simulink model "s_c107m32k_vlbi"  (R2018a)
settings: Solver=VariableStepDiscrete  StartTime=0.0  StopTime=(2^15)*10  RelTol=1e-3
undefined symbols (not defined in the file): fft_stages, n_bits_xengs
libraries: xbsIndex_r4 x23049, casper_library_misc x45, xps_library x4, casper_library_scopes x3, simulink x2
(part 44 of 201)

== system s_c107m32k_vlbi/bs_delay1/bus_expand1 ==
  bus_in : Inport
  reinterpret1 : xbsIndex_r4/Reinterpret  force_arith_type=on  arith_type="Signed  (2's comp)"  force_bin_pt=on  bin_pt=31  block_type=reinterpret
  reinterpret2 : xbsIndex_r4/Reinterpret  force_arith_type=on  arith_type="Signed  (2's comp)"  force_bin_pt=on  bin_pt=31  block_type=reinterpret
  reinterpret3 : xbsIndex_r4/Reinterpret  force_arith_type=on  arith_type="Signed  (2's comp)"  force_bin_pt=on  bin_pt=31  block_type=reinterpret
  reinterpret4 : xbsIndex_r4/Reinterpret  force_arith_type=on  arith_type=Unsigned  force_bin_pt=on  bin_pt=32  block_type=reinterpret
  slice1 : xbsIndex_r4/Slice  nbits=32  boolean_output=off  mode=Upper Bit Location + Width  bit1=-128  base1=MSB of Input  bit0=0  base0=LSB of Input  dbl_ovrd=off  block_type=slice
  slice2 : xbsIndex_r4/Slice  nbits=32  boolean_output=off  mode=Upper Bit Location + Width  bit1=-96  base1=MSB of Input  bit0=0  base0=LSB of Input  dbl_ovrd=off  block_type=slice
  slice3 : xbsIndex_r4/Slice  nbits=32  boolean_output=off  mode=Upper Bit Location + Width  bit1=-64  base1=MSB of Input  bit0=0  base0=LSB of Input  dbl_ovrd=off  block_type=slice
  slice4 : xbsIndex_r4/Slice  nbits=64  boolean_output=off  mode=Upper Bit Location + Width  bit1=0  base1=MSB of Input  bit0=0  base0=LSB of Input  dbl_ovrd=off  block_type=slice
  msb_out4 : Outport
  out3 : Outport  Port=2
  out2 : Outport  Port=3
  lsb_out1 : Outport  Port=4
  wires:
  reinterpret1/1 -> lsb_out1/1
  slice1/1 -> reinterpret1/1
  reinterpret2/1 -> out2/1
  slice2/1 -> reinterpret2/1
  reinterpret3/1 -> out3/1
  slice3/1 -> reinterpret3/1
  reinterpret4/1 -> msb_out4/1
  slice4/1 -> reinterpret4/1
  bus_in/1 -> slice1/1, slice2/1, slice3/1, slice4/1

== system s_c107m32k_vlbi/bs_delay1/delay_gen ==
  note: coarse delay rotates phase around 0th
      | channel. We want to reference with respect to
      | centre of band. So subtract half the coarse
      | delay amount.
  note: Extract fractional part
  note: Extract whole part
  note: Need negative slope
      | for positive deay
  note: Make space here (cast) for the upcoming
      | scaling, ensuring that we keep the
      | required precision.
      | Shift phase and delay rates down
      | to fit into specified range.
      | An update is only done at the end of
      | every FFT spectrum so modify shift to
      | not be as large
  sync_in : Inport
  init : Inport  Port=2
  din : Inport  Port=3
  idx_in : Inport  Port=4
  den : Inport  Port=5
  load : Inport  Port=6
  phase : Inport  Port=7
  d/dt_phase : Inport  Port=8
  delay : Inport  Port=9
  d/dt_delay : Inport  Port=10
  invert_slope : Inport  Port=11
  AddSub : xbsIndex_r4/AddSub  mode=Addition  use_carryin=off  use_carryout=off  en=off  latency=1  precision=Full  arith_type=Unsigned  n_bits=16  bin_pt=14  quantization=Truncate  overflow=Wrap  use_behavioral_HDL=on  hw_selection=Fabric  pipelined=off  dbl_ovrd=off  block_type=addsub
  Concat : xbsIndex_r4/Concat  num_inputs=4  dbl_ovrd=off  block_type=concat
  Constant : xbsIndex_r4/Constant  const=1  gui_display_data_type=Fixed-point  arith_type=Unsigned  n_bits=1  bin_pt=0  preci_type=Single  exp_width=8  frac_width=24  explicit_period=on  period=1  equ=P=C  opselect=C  inp2=PCIN>>17  opr=+  inp1=P  carry=CIN  dbl_ovrd=off  block_type=constant
  Convert : xbsIndex_r4/Convert  gui_display_data_type=Fixed-point  arith_type="Signed  (2's comp)"  n_bits=comp_phase_rate_bits  bin_pt=comp_phase_rate_bin_pt  float_type=Single  exp_bits=8  fraction_bits=24  quantization="Round  (unbiased: +/- Inf)"  overflow=Saturate  en=off  latency=0  pipeline=off  dbl_ovrd=off  block_type=convert
  Convert1 : xbsIndex_r4/Convert  gui_display_data_type=Fixed-point  arith_type="Signed  (2's comp)"  n_bits=comp_delay_rate_bits  bin_pt=comp_delay_rate_bin_pt  float_type=Single  exp_bits=8  fraction_bits=24  quantization="Round  (unbiased: +/- Inf)"  overflow=Saturate  en=off  latency=0  pipeline=off  dbl_ovrd=off  block_type=convert
  Convert4 : xbsIndex_r4/Convert  gui_display_data_type=Fixed-point  arith_type="Signed  (2's comp)"  n_bits=max(phase_bits, comp_phase_rate_bits)  bin_pt=max(phase_bits-1, comp_phase_rate_bin_pt)  float_type=Single  exp_bits=8  fraction_bits=24  quantization=Truncate  overflow=Wrap  en=off  latency=1  pipeline=on  dbl_ovrd=off  block_type=convert
      settings: block_version=10.1.3
  Convert5 : xbsIndex_r4/Convert  gui_display_data_type=Fixed-point  arith_type=Unsigned  n_bits=cd_bits  bin_pt=0  float_type=Single  exp_bits=8  fraction_bits=24  quantization=Truncate  overflow=Wrap  en=off  latency=1  pipeline=on  dbl_ovrd=off  block_type=convert
      settings: block_version=10.1.3
  Convert6 : xbsIndex_r4/Convert  gui_display_data_type=Fixed-point  arith_type=Unsigned  n_bits=max(delay_bin_pt, comp_delay_rate_bin_pt)  bin_pt=max(delay_bin_pt, comp_delay_rate_bin_pt)  float_type=Single  exp_bits=8  fraction_bits=24  quantization=Truncate  overflow=Wrap  en=off  latency=1  pipeline=on  dbl_ovrd=off  block_type=convert
      settings: block_version=10.1.3
  Delay{1..14,16} (15 alike) : xbsIndex_r4/Delay  rst=off  infoeditControl=Selection of Reset will increase slice count due to use of real FFs and instead of SRLs  en=off  latency=1  reg_retiming=on  dbl_ovrd=off  block_type=delay
      settings: block_version=11.4
  Mux : xbsIndex_r4/Mux  inputs=2  en=off  latency=1  precision=Full  arith_type=Unsigned  n_bits=16  bin_pt=14  quantization=Truncate  overflow=Wrap  dbl_ovrd=off  block_type=mux
      settings: block_version=11.4
  Negate : xbsIndex_r4/Negate  precision=Full  arith_type="Signed  (2's comp)"  n_bits=lookup_bits + fft_len  bin_pt=lookup_bits + fft_len - 1  quantization=Truncate  overflow=Saturate  en=off  latency=1  dbl_ovrd=off  block_type=negate
      settings: block_version=11.4
  Reinterpret{,1..3} (4 alike) : xbsIndex_r4/Reinterpret  force_arith_type=on  arith_type=Unsigned  force_bin_pt=on  bin_pt=0  block_type=reinterpret
  Slice5 : xbsIndex_r4/Slice  nbits=2  boolean_output=off  mode=Lower Bit Location + Width  bit1=0  base1=MSB of Input  bit0=0  base0=LSB of Input  dbl_ovrd=off  block_type=slice
  Terminator : Terminator
  Terminator1 : Terminator
  bus_expand : Subsystem  AncestorBlock=casper_library_flow_control/bus_expand  mask(bus_expand){mode=divisions of arbitrary size, outputNum=1, outputWidth=[1 1 data_bits n_bits_index], outputBinaryPt=[0 0 0 0], outputArithmeticType=[2 2 0 0], show_format=off, outputToWorkspace=off, variablePrefix=out, outputToModelAsWell=on}
      mask prompts: outputNum "Number of outputs:"; outputWidth "Output width [msb ... lsb]:"; outputBinaryPt "Output binary point position [msb ... lsb]:"; outputArithmeticType "Output arithmetic type (ufix=0, fix=1, bool=2) [msb ... lsb]:"; show_format "Print format string?"; outputToWorkspace "Output to workspace?"; variablePrefix "Variable name prefix:"; outputToModelAsWell "Output to model as well?"
      mask help:
      | Expands a 'bus' made using a bus_create or Xilinx
      | concat block.
      | The input will be divided into the specified number
      | of outputs with the specified arithmetic types.
      | Divisions are made from most significant bit.
      mask init: same as s_c107m32k_vlbi/bus_expand1
      settings: AttributesFormatString=4 outputs
      mask TypeOptions mode: divisions of equal size | divisions of arbitrary size
      mask Callback mode: bus_expand_callback();
      mask Callback outputWidth: bus_expand_callback();
      mask Callback outputToWorkspace: bus_expand_callback();
  delay_calc : Subsystem  mask{bit_width=max(delay_bits, comp_delay_rate_bits), bin_pt=max(delay_bin_pt, comp_delay_rate_bin_pt)}
      mask prompts: bit_width "Coefficient bit width"; bin_pt "Coefficient binary point"
  half_cd : xbsIndex_r4/Shift  shift_dir=Right  shift_bits=1  en=off  latency=0  precision=User Defined  arith_type=Unsigned  n_bits=2  bin_pt=1  quantization=Truncate  overflow=Saturate  dbl_ovrd=off  block_type=shift
  normalise+fft0 : xbsIndex_r4/Shift  shift_dir=Right  shift_bits=phase_rate_scale_factor  en=off  latency=0  precision=Full  arith_type="Signed  (2's comp)"  n_bits=comp_phase_rate_bits  bin_pt=comp_phase_rate_bin_pt  quantization="Round  (unbiased: +/- Inf)"  overflow=Saturate  dbl_ovrd=off  block_type=shift
  normalise+fft1 : xbsIndex_r4/Shift  shift_dir=Right  shift_bits=delay_rate_scale_factor  en=off  latency=0  precision=Full  arith_type="Signed  (2's comp)"  n_bits=comp_delay_rate_bits  bin_pt=comp_delay_rate_bin_pt  quantization="Round  (unbiased: +/- Inf)"  overflow=Saturate  dbl_ovrd=off  block_type=shift
  phase_calc : Subsystem  mask{bit_width=max(phase_bits, comp_phase_rate_bits), bin_pt=max(phase_bits-1, comp_phase_rate_bin_pt)}
      mask prompts: bit_width "Coefficient bit width"; bin_pt "Coefficient binary point"
  sync_out : Outport
  dout : Outport  Port=2
  idx_out : Outport  Port=3
  dvalid : Outport  Port=4
  cd_o : Outport  Port=5
  slope_out : Outport  Port=6
  phase_out : Outport  Port=7
  load_out : Outport  Port=8
  wires:
  Convert1/1 -> normalise+fft1/1
  Convert/1 -> normalise+fft0/1
  Delay14/1 -> cd_o/1
  Delay10/1 -> phase_out/1
  Delay7/1 -> load_out/1
  Delay6/1 -> bus_expand/1(bus_in)
  bus_expand/4(lsb_out1) -> idx_out/1
  bus_expand/3(out2) -> dout/1
  bus_expand/2(out3) -> dvalid/1
  idx_in/1 -> Reinterpret3/1
  din/1 -> Reinterpret2/1
  den/1 -> Reinterpret1/1
  bus_expand/1(msb_out4) -> sync_out/1
  Reinterpret3/1 -> Concat/4
  Reinterpret2/1 -> Concat/3
  Reinterpret1/1 -> Concat/2
  Reinterpret/1 -> Concat/1
  Delay13/1 -> Mux/3
  delay_calc/1(dout) -> Terminator1/1
  Constant/1 -> delay_calc/1(din)
  delay/1 -> delay_calc/2(val)
  phase/1 -> phase_calc/2(val)
  Delay12/1 -> Convert6/1
  Delay11/1 -> Delay8/1
  Delay3/1 -> AddSub/1
  Delay1/1 -> Delay4/1
  Delay9/1 -> Delay6/1
  phase_calc/1(dout) -> Delay11/1
  AddSub/1 -> Convert4/1
  phase_calc/2(coeff) -> Delay3/1
  half_cd/1 -> AddSub/2
  Slice5/1 -> half_cd/1
  Convert5/1 -> Delay5/1, Slice5/1
  Concat/1 -> phase_calc/1(din)
  sync_in/1 -> Reinterpret/1
  init/1 -> [tick]
  Delay8/1 -> Delay9/1
  Negate/1 -> Mux/2
  invert_slope/1 -> Mux/1
  Delay5/1 -> Delay16/1
  Delay4/1 -> Delay2/1
  load/1 -> [en]
  normalise+fft0/1 -> phase_calc/3(val_inc)
  [en] -> phase_calc/4(en)
  [en] -> delay_calc/4(en)
  [tick] -> phase_calc/5(update)
  [tick] -> delay_calc/5(update)
  delay_calc/2(coeff) -> Convert5/1, Delay12/1
  phase_calc/3(en_o) -> Delay1/1
  delay_calc/3(en_o) -> Terminator/1
  Convert6/1 -> Negate/1, Delay13/1
  Mux/1 -> slope_out/1
  Convert4/1 -> Delay10/1
  Delay2/1 -> Delay7/1
  Delay16/1 -> Delay14/1
  d/dt_phase/1 -> Convert/1
  normalise+fft1/1 -> delay_calc/3(val_inc)
  d/dt_delay/1 -> Convert1/1

== system s_c107m32k_vlbi/bs_delay1/edge_detect ==
  in : Inport
  Delay : xbsIndex_r4/Delay  rst=off  infoeditControl=Selection of Reset will increase slice count due to use of real FFs and instead of SRLs  en=off  latency=1  reg_retiming=off  dbl_ovrd=off  block_type=delay
      settings: xl_area=[0, 0, 0, 0, 0, 0, 0]
  Inverter : xbsIndex_r4/Inverter  en=off  latency=0  dbl_ovrd=off  block_type=inv
      settings: xl_area=[0, 0, 0, 0, 0, 0, 0]
  edge_op : xbsIndex_r4/Logical  logical_function=NOR  inputs=2  en=off  latency=0  precision=Full  arith_type=Unsigned  n_bits=8  bin_pt=2  align_bp=on  dbl_ovrd=off  block_type=logical
      settings: xl_area=[0, 0, 0, 0, 0, 0, 0]
  out : Outport
  wires:
  Delay/1 -> edge_op/2
  in/1 -> Delay/1, Inverter/1
  edge_op/1 -> out/1
  Inverter/1 -> edge_op/1

== system s_c107m32k_vlbi/bs_delay1/generate_pkt_sync1 ==
  sync : Inport
  valid : Inport  Port=2
  data : Inport  Port=3
  Constant : xbsIndex_r4/Constant  const=(2^pktlen_bits)-1  gui_display_data_type=Fixed-point  arith_type=Unsigned  n_bits=pktlen_bits  bin_pt=0  preci_type=Single  exp_width=8  frac_width=24  explicit_period=on  period=1  equ=P=C  opselect=C  inp2=PCIN>>17  opr=+  inp1=P  carry=CIN  dbl_ovrd=off  block_type=constant
  Counter1 : xbsIndex_r4/Counter  cnt_type=Free Running  cnt_to=Inf  operation=Up  start_count=0  cnt_by_val=1  arith_type=Unsigned  n_bits=pktlen_bits  bin_pt=0  load_pin=off  rst=on  en=on  explicit_period=on  period=1  use_behavioral_HDL=on  implementation=Fabric  dbl_ovrd=off  block_type=counter
  Delay{,1..5} (6 alike) : xbsIndex_r4/Delay  rst=off  infoeditControl=Selection of Reset will increase slice count due to use of real FFs and instead of SRLs  en=off  latency=1  reg_retiming=on  dbl_ovrd=off  block_type=delay
  Logical : xbsIndex_r4/Logical  logical_function=OR  inputs=2  en=off  latency=1  precision=Full  arith_type=Unsigned  n_bits=16  bin_pt=0  align_bp=on  dbl_ovrd=off  block_type=logical
  Logical1 : xbsIndex_r4/Logical  logical_function=AND  inputs=2  en=off  latency=0  precision=Full  arith_type=Unsigned  n_bits=16  bin_pt=0  align_bp=on  dbl_ovrd=off  block_type=logical
  Relational : xbsIndex_r4/Relational  mode=a=b  op_type=Bool  en=off  latency=1  dbl_ovrd=off  block_type=relational
  pipeline1 : Subsystem  Tag=cmac_delinked  mask(pipeline){csp_latency=2}
      mask prompts: csp_latency "Latency"
      mask help:
      | An explicitly laid-out delay line to avoid mapping to SRL16s
      | for use in pipelining to help achieve timing closure.
      mask init:
      | pipeline_init(gcb,'latency',csp_latency);
      settings: AttributesFormatString=Latency = %<latency>
      mask Display:
      | port_label('input', 1, 'd');
      | port_label('output', 1, 'q');
      | disp(['Z^-', num2str(csp_latency)]);
  pipeline2 : Subsystem  Tag=cmac_delinked  mask(pipeline){csp_latency=2}
      mask prompts: csp_latency "Latency"
      mask help:
      | An explicitly laid-out delay line to avoid mapping to SRL16s
      | for use in pipelining to help achieve timing closure.
      mask init:
      | pipeline_init(gcb,'latency',csp_latency);
      settings: AttributesFormatString=Latency = %<latency>
      mask Display:
      | port_label('input', 1, 'd');
      | port_label('output', 1, 'q');
      | disp(['Z^-', num2str(csp_latency)]);
  pipeline24 : Subsystem  Tag=cmac_delinked  mask(pipeline){csp_latency=2}
      mask prompts: csp_latency "Latency"
      mask help:
      | An explicitly laid-out delay line to avoid mapping to SRL16s
      | for use in pipelining to help achieve timing closure.
      mask init:
      | pipeline_init(gcb,'latency',csp_latency);
      settings: AttributesFormatString=Latency = %<latency>
      mask Display:
      | port_label('input', 1, 'd');
      | port_label('output', 1, 'q');
      | disp(['Z^-', num2str(csp_latency)]);
  out_sync : Outport
  out_valid : Outport  Port=2
  out_data : Outport  Port=3
  packet_sync : Outport  Port=4
  wires:
  Delay5/1 -> Logical1/1, Delay/1
  Delay4/1 -> Delay1/1, Logical/1
  Delay3/1 -> Delay2/1
  Logical/1 -> packet_sync/1
  Delay/1 -> out_valid/1
  Delay1/1 -> out_sync/1
  Delay2/1 -> out_data/1
  pipeline2/1(q) -> Counter1/1, Delay4/1
  pipeline1/1(q) -> Counter1/2, Delay5/1
  pipeline24/1(q) -> Delay3/1
  data/1 -> pipeline24/1(d)
  valid/1 -> pipeline1/1(d)
  sync/1 -> pipeline2/1(d)
  Logical1/1 -> Logical/2  "ns"
  Relational/1 -> Logical1/2
  Constant/1 -> Relational/2
  Counter1/1 -> Relational/1  "pkt_counter"

== system s_c107m32k_vlbi/bs_delay1/mangled_dwp ==
  note: JRM: customised block
      | Replaced BRAM delays
      | with distributed memory.
      | THIS BLOCK IS NO LONGER PROPERLY PARAMETERISED!
  sync : Inport
  delay : Inport  Port=2
  ld_delay : Inport  Port=3
  data_in0 : Inport  Port=4
  data_in1 : Inport  Port=5
  data_in2 : Inport  Port=6
  data_in3 : Inport  Port=7
  data_in4 : Inport  Port=8
  data_in5 : Inport  Port=9
  data_in6 : Inport  Port=10
  data_in7 : Inport  Port=11
  en : Inport  Port=12
  AddSub{1..7} (7 alike) : xbsIndex_r4/AddSub  mode=Addition  use_carryin=off  use_carryout=off  en=off  latency=0  precision=Full  arith_type=Unsigned  n_bits=1  bin_pt=0  quantization=Truncate  overflow=Wrap  use_behavioral_HDL=off  hw_selection=Fabric  pipelined=off  dbl_ovrd=off  block_type=addsub
  Constant1 : xbsIndex_r4/Constant  const=6  gui_display_data_type=Fixed-point  arith_type=Unsigned  n_bits=3  bin_pt=0  preci_type=Single  exp_width=8  frac_width=24  explicit_period=on  period=1  equ=P=C  opselect=C  inp2=PCIN>>17  opr=+  inp1=P  carry=CIN  dbl_ovrd=off  block_type=constant
  Constant2 : xbsIndex_r4/Constant  const=5  gui_display_data_type=Fixed-point  arith_type=Unsigned  n_bits=3  bin_pt=0  preci_type=Single  exp_width=8  frac_width=24  explicit_period=on  period=1  equ=P=C  opselect=C  inp2=PCIN>>17  opr=+  inp1=P  carry=CIN  dbl_ovrd=off  block_type=constant
  Constant3 : xbsIndex_r4/Constant  const=4  gui_display_data_type=Fixed-point  arith_type=Unsigned  n_bits=3  bin_pt=0  preci_type=Single  exp_width=8  frac_width=24  explicit_period=on  period=1  equ=P=C  opselect=C  inp2=PCIN>>17  opr=+  inp1=P  carry=CIN  dbl_ovrd=off  block_type=constant
  Constant4 : xbsIndex_r4/Constant  const=3  gui_display_data_type=Fixed-point  arith_type=Unsigned  n_bits=3  bin_pt=0  preci_type=Single  exp_width=8  frac_width=24  explicit_period=on  period=1  equ=P=C  opselect=C  inp2=PCIN>>17  opr=+  inp1=P  carry=CIN  dbl_ovrd=off  block_type=constant
  Constant5 : xbsIndex_r4/Constant  const=2  gui_display_data_type=Fixed-point  arith_type=Unsigned  n_bits=3  bin_pt=0  preci_type=Single  exp_width=8  frac_width=24  explicit_period=on  period=1  equ=P=C  opselect=C  inp2=PCIN>>17  opr=+  inp1=P  carry=CIN  dbl_ovrd=off  block_type=constant
  Constant6 : xbsIndex_r4/Constant  const=1  gui_display_data_type=Fixed-point  arith_type=Unsigned  n_bits=3  bin_pt=0  preci_type=Single  exp_width=8  frac_width=24  explicit_period=on  period=1  equ=P=C  opselect=C  inp2=PCIN>>17  opr=+  inp1=P  carry=CIN  dbl_ovrd=off  block_type=constant
  Constant7 : xbsIndex_r4/Constant  const=0  gui_display_data_type=Fixed-point  arith_type=Unsigned  n_bits=3  bin_pt=0  preci_type=Single  exp_width=8  frac_width=24  explicit_period=on  period=1  equ=P=C  opselect=C  inp2=PCIN>>17  opr=+  inp1=P  carry=CIN  dbl_ovrd=off  block_type=constant
  Convert{1..7} (7 alike) : xbsIndex_r4/Convert  gui_display_data_type=Fixed-point  arith_type=Unsigned  n_bits=1  bin_pt=0  float_type=Single  exp_bits=8  fraction_bits=24  quantization=Truncate  overflow=Wrap  en=off  latency=0  pipeline=off  dbl_ovrd=off  block_type=convert
  Relational{1..7} (7 alike) : xbsIndex_r4/Relational  mode=a>b  op_type=Bool  en=off  latency=0  dbl_ovrd=off  block_type=relational
  barrel_switcher : Subsystem  mask(barrel_switcher){n_inputs=3, async=on}
      mask prompts: n_inputs "Number of Inputs: (2^?)"; async "Asynchronous operation"
      mask help:
      | Shifts input to right by amount specified on sel,
      | wrapping around into higher order bits.
      mask init:
      | barrel_switcher_init(gcb,...
      |     'n_inputs', n_inputs, ...
      |     'async', async);
      mask Help: eval('xlWeb(''http://casper.berkeley.edu/wiki/Barrel_switcher'')')
  bram_rd_addrs : xbsIndex_r4/Slice  nbits=1  boolean_output=off  mode=Lower Bit Location + Width  bit1=0  base1=MSB of Input  bit0=3  base0=LSB of Input  dbl_ovrd=off  block_type=slice
  delay_dp0 : Subsystem  mask(delay_bram_prog_dp){ram_bits=2, bram_latency=3, async=on}
      mask prompts: ram_bits "Max delay (2^?)"; bram_latency "BRAM latency"; async "asynchronous operation"
      mask init:
      | %delay_bram_prog_dp_init(gcb, ...
      | %    'ram_bits', ram_bits, ...
      | %    'bram_latency', bram_latency, ...
      | %    'async', async);
  delay_dp1 : Subsystem  mask(delay_bram_prog_dp){ram_bits=2, bram_latency=3, async=on}
      mask prompts: ram_bits "Max delay (2^?)"; bram_latency "BRAM latency"; async "asynchronous operation"
      mask init:
      | %delay_bram_prog_dp_init(gcb, ...
      | %    'ram_bits', ram_bits, ...
      | %    'bram_latency', bram_latency, ...
      | %    'async', async);
  delay_dp2 : Subsystem  mask(delay_bram_prog_dp){ram_bits=2, bram_latency=3, async=on}
      mask prompts: ram_bits "Max delay (2^?)"; bram_latency "BRAM latency"; async "asynchronous operation"
      mask init:
      | %delay_bram_prog_dp_init(gcb, ...
      | %    'ram_bits', ram_bits, ...
      | %    'bram_latency', bram_latency, ...
      | %    'async', async);
  delay_dp3 : Subsystem  mask(delay_bram_prog_dp){ram_bits=2, bram_latency=3, async=on}
      mask prompts: ram_bits "Max delay (2^?)"; bram_latency "BRAM latency"; async "asynchronous operation"
      mask init:
      | %delay_bram_prog_dp_init(gcb, ...
      | %    'ram_bits', ram_bits, ...
      | %    'bram_latency', bram_latency, ...
      | %    'async', async);
  delay_dp4 : Subsystem  mask(delay_bram_prog_dp){ram_bits=2, bram_latency=3, async=on}
      mask prompts: ram_bits "Max delay (2^?)"; bram_latency "BRAM latency"; async "asynchronous operation"
      mask init:
      | %delay_bram_prog_dp_init(gcb, ...
      | %    'ram_bits', ram_bits, ...
      | %    'bram_latency', bram_latency, ...
      | %    'async', async);
  delay_dp5 : Subsystem  mask(delay_bram_prog_dp){ram_bits=2, bram_latency=3, async=on}
      mask prompts: ram_bits "Max delay (2^?)"; bram_latency "BRAM latency"; async "asynchronous operation"
      mask init:
      | %delay_bram_prog_dp_init(gcb, ...
      | %    'ram_bits', ram_bits, ...
      | %    'bram_latency', bram_latency, ...
      | %    'async', async);
  delay_dp6 : Subsystem  mask(delay_bram_prog_dp){ram_bits=2, bram_latency=3, async=on}
      mask prompts: ram_bits "Max delay (2^?)"; bram_latency "BRAM latency"; async "asynchronous operation"
      mask init:
      | %delay_bram_prog_dp_init(gcb, ...
      | %    'ram_bits', ram_bits, ...
      | %    'bram_latency', bram_latency, ...
      | %    'async', async);
  delay_dp7 : Subsystem  mask(delay_bram_prog_dp){ram_bits=2, bram_latency=3, async=on}
      mask prompts: ram_bits "Max delay (2^?)"; bram_latency "BRAM latency"; async "asynchronous operation"
      mask init:
      | %delay_bram_prog_dp_init(gcb, ...
      | %    'ram_bits', ram_bits, ...
      | %    'bram_latency', bram_latency, ...
      | %    'async', async);
  delay_reg : xbsIndex_r4/Register  init=0  rst=off  en=on  dbl_ovrd=off  block_type=register
  delay_sel : xbsIndex_r4/Delay  rst=off  infoeditControl=Selection of Reset will increase slice count due to use of real FFs and instead of SRLs  en=off  latency=4  reg_retiming=on  dbl_ovrd=off  block_type=delay
  en_delay0 : xbsIndex_r4/Delay  rst=off  infoeditControl=Selection of Reset will increase slice count due to use of real FFs and instead of SRLs  en=off  latency=0  reg_retiming=on  dbl_ovrd=off  block_type=delay
  en_delay1 : xbsIndex_r4/Delay  rst=off  infoeditControl=Selection of Reset will increase slice count due to use of real FFs and instead of SRLs  en=off  latency=4  reg_retiming=on  dbl_ovrd=off  block_type=delay
  shift_sel : xbsIndex_r4/Slice  nbits=3  boolean_output=off  mode=Lower Bit Location + Width  bit1=0  base1=MSB of Input  bit0=0  base0=LSB of Input  dbl_ovrd=off  block_type=slice
  sync_delay : xbsIndex_r4/Delay  rst=off  infoeditControl=Selection of Reset will increase slice count due to use of real FFs and instead of SRLs  en=off  latency=4  reg_retiming=on  dbl_ovrd=off  block_type=delay
  sync_out : Outport
  data_out0 : Outport  Port=2
  data_out1 : Outport  Port=3
  data_out2 : Outport  Port=4
  data_out3 : Outport  Port=5
  data_out4 : Outport  Port=6
  data_out5 : Outport  Port=7
  data_out6 : Outport  Port=8
  data_out7 : Outport  Port=9
  dvalid : Outport  Port=10
  wires:
  AddSub7/1 -> delay_dp7/2(delay)  "dp7"
  Convert7/1 -> AddSub7/2
  Relational7/1 -> Convert7/1
  Constant7/1 -> Relational7/2
  delay_dp7/1(dout) -> barrel_switcher/3(In1)
  data_in7/1 -> delay_dp7/1(din)  "dp_val7"
  AddSub6/1 -> delay_dp6/2(delay)  "dp6"
  Convert6/1 -> AddSub6/2
  Relational6/1 -> Convert6/1
  Constant6/1 -> Relational6/2
  delay_dp6/1(dout) -> barrel_switcher/4(In2)
  data_in6/1 -> delay_dp6/1(din)  "dp_val6"
  AddSub5/1 -> delay_dp5/2(delay)  "dp5"
  Convert5/1 -> AddSub5/2
  Relational5/1 -> Convert5/1
  Constant5/1 -> Relational5/2
  delay_dp5/1(dout) -> barrel_switcher/5(In3)
  data_in5/1 -> delay_dp5/1(din)  "dp_val5"
  AddSub4/1 -> delay_dp4/2(delay)  "dp4"
  Convert4/1 -> AddSub4/2
  Relational4/1 -> Convert4/1
  Constant4/1 -> Relational4/2
  delay_dp4/1(dout) -> barrel_switcher/6(In4)
  data_in4/1 -> delay_dp4/1(din)  "dp_val4"
  AddSub3/1 -> delay_dp3/2(delay)  "dp3"
  Convert3/1 -> AddSub3/2
  Relational3/1 -> Convert3/1
  Constant3/1 -> Relational3/2
  delay_dp3/1(dout) -> barrel_switcher/7(In5)
  data_in3/1 -> delay_dp3/1(din)  "dp_val3"
  AddSub2/1 -> delay_dp2/2(delay)  "dp2"
  Convert2/1 -> AddSub2/2
  Relational2/1 -> Convert2/1
  Constant2/1 -> Relational2/2
  delay_dp2/1(dout) -> barrel_switcher/8(In6)
  data_in2/1 -> delay_dp2/1(din)  "dp_val2"
  AddSub1/1 -> delay_dp1/2(delay)  "dp1"
  Convert1/1 -> AddSub1/2
  Relational1/1 -> Convert1/1
  Constant1/1 -> Relational1/2
  delay_dp1/1(dout) -> barrel_switcher/9(In7)
  data_in1/1 -> delay_dp1/1(din)  "dp_val1"
  bram_rd_addrs/1 -> AddSub7/1, AddSub6/1, AddSub5/1, AddSub4/1, AddSub3/1, AddSub2/1, AddSub1/1, delay_dp0/2(delay)  "dp0"
  delay_dp0/1(dout) -> barrel_switcher/10(In8)
  data_in0/1 -> delay_dp0/1(din)  "dp_val0"
  barrel_switcher/2(Out1) -> data_out7/1
  barrel_switcher/3(Out2) -> data_out6/1
  barrel_switcher/4(Out3) -> data_out5/1
  barrel_switcher/5(Out4) -> data_out4/1
  barrel_switcher/6(Out5) -> data_out3/1
  barrel_switcher/7(Out6) -> data_out2/1
  barrel_switcher/8(Out7) -> data_out1/1
  barrel_switcher/9(Out8) -> data_out0/1
  delay_sel/1 -> barrel_switcher/1(sel)
  shift_sel/1 -> Relational7/1, Relational6/1, Relational5/1, Relational4/1, Relational3/1, Relational2/1, Relational1/1, delay_sel/1
  barrel_switcher/10(dvalid) -> dvalid/1
  en_delay1/1 -> barrel_switcher/11(en)
  barrel_switcher/1(sync_out) -> sync_out/1
  sync_delay/1 -> barrel_switcher/2(sync_in)
  delay_reg/1 -> shift_sel/1, bram_rd_addrs/1
  ld_delay/1 -> delay_reg/2
  delay/1 -> delay_reg/1
  sync/1 -> sync_delay/1
  en_delay0/1 -> delay_dp0/3(en), en_delay1/1, delay_dp1/3(en), delay_dp2/3(en), delay_dp7/3(en), delay_dp6/3(en), delay_dp4/3(en), delay_dp3/3(en), delay_dp5/3(en)  "dp_en"
  en/1 -> en_delay0/1

== system s_c107m32k_vlbi/bs_delay1/pipeline1 ==
  d : Inport
  Register0 : xbsIndex_r4/Register  init=0  rst=off  en=off  dbl_ovrd=off  block_type=register
      settings: block_version=11.4
  Register1 : xbsIndex_r4/Register  init=0  rst=off  en=off  dbl_ovrd=off  block_type=register
      settings: block_version=11.4
  q : Outport
  wires:
  Register1/1 -> q/1
  d/1 -> Register0/1
  Register0/1 -> Register1/1

== system s_c107m32k_vlbi/bs_delay1/pipeline2 ==
  d : Inport
  Register0 : xbsIndex_r4/Register  init=0  rst=off  en=off  dbl_ovrd=off  block_type=register
      settings: block_version=11.4
  Register1 : xbsIndex_r4/Register  init=0  rst=off  en=off  dbl_ovrd=off  block_type=register
      settings: block_version=11.4
  q : Outport
  wires:
  Register1/1 -> q/1
  d/1 -> Register0/1
  Register0/1 -> Register1/1

== system s_c107m32k_vlbi/bs_delay1/pipeline3 ==
  d : Inport
  Register0 : xbsIndex_r4/Register  init=0  rst=off  en=off  dbl_ovrd=off  block_type=register
      settings: block_version=11.4
  Register1 : xbsIndex_r4/Register  init=0  rst=off  en=off  dbl_ovrd=off  block_type=register
      settings: block_version=11.4
  q : Outport
  wires:
  Register0/1 -> Register1/1
  d/1 -> Register0/1
  Register1/1 -> q/1

== system s_c107m32k_vlbi/bs_delay1/pipeline33 ==
  d : Inport
  Register0 : xbsIndex_r4/Register  init=0  rst=off  en=off  dbl_ovrd=off  block_type=register
      settings: block_version=11.4
  Register1 : xbsIndex_r4/Register  init=0  rst=off  en=off  dbl_ovrd=off  block_type=register
      settings: block_version=11.4
  q : Outport
  wires:
  Register0/1 -> Register1/1
  d/1 -> Register0/1
  Register1/1 -> q/1

== system s_c107m32k_vlbi/bs_delay1/req_delay ==
  out_reg : Inport
  assert_reg : xbsIndex_r4/Assert  assert_type=on  type_source=Explicitly  gui_display_data_type=Fixed-point  arith_type=Unsigned  n_bits=4  bin_pt=0  preci_type=Single  exp_width=8  frac_width=24  assert_rate=off  rate_source=Explicitly  period=1  output_port=on  block_type=assert
  cast_gw : xbsIndex_r4/Convert  gui_display_data_type=Fixed-point  arith_type=Unsigned  n_bits=32  bin_pt=0  float_type=Single  exp_bits=8  fraction_bits=24  quantization=Truncate  overflow=Wrap  en=off  latency=1  pipeline=off  dbl_ovrd=off  block_type=convert
  io_delay : xbsIndex_r4/Delay  rst=off  infoeditControl=Selection of Reset will increase slice count due to use of real FFs and instead of SRLs  en=off  latency=0  reg_retiming=on  dbl_ovrd=off  block_type=delay
  reint1 : xbsIndex_r4/Reinterpret  force_arith_type=on  arith_type=Unsigned  force_bin_pt=on  bin_pt=0  block_type=reinterpret
  s_c107m32k_vlbi_bs_delay1_req_delay_user_data_in : xbsIndex_r4/Gateway Out  inherit_from_input=off  hdl_port=on  rows=1  columns=1  UseAsDAC=off  DACChannel='1'  interface=None  automatic_assignment=on  address_offset=hex2dec('00')  intf_name=''  intf_description=''  timing_constraint=None  locs_specified=off  LOCs={}  io_standard={}  block_type=gatewayout
  sim_out : Terminator
  wires:
  io_delay/1 -> cast_gw/1
  cast_gw/1 -> s_c107m32k_vlbi_bs_delay1_req_delay_user_data_in/1
  s_c107m32k_vlbi_bs_delay1_req_delay_user_data_in/1 -> sim_out/1
  out_reg/1 -> assert_reg/1
  assert_reg/1 -> reint1/1
  reint1/1 -> io_delay/1

== system s_c107m32k_vlbi/bs_delay1/snap_bs_in ==
  in_data : Inport
  in_ts : Inport  Port=2
  in_ld : Inport  Port=3
  in_delay : Inport  Port=4
  in_valid : Inport  Port=5
  we : Inport  Port=6
  trig : Inport  Port=7
  assert_data : xbsIndex_r4/Assert  assert_type=on  type_source=Explicitly  gui_display_data_type=Fixed-point  arith_type=Unsigned  n_bits=48  bin_pt=0  preci_type=Single  exp_width=8  frac_width=24  assert_rate=off  rate_source=Explicitly  period=1  output_port=on  block_type=assert
  assert_delay : xbsIndex_r4/Assert  assert_type=on  type_source=Explicitly  gui_display_data_type=Fixed-point  arith_type=Unsigned  n_bits=4  bin_pt=0  preci_type=Single  exp_width=8  frac_width=24  assert_rate=off  rate_source=Explicitly  period=1  output_port=on  block_type=assert
  assert_ld : xbsIndex_r4/Assert  assert_type=on  type_source=Explicitly  gui_display_data_type=Boolean  arith_type=Boolean  n_bits=1  bin_pt=0  preci_type=Single  exp_width=8  frac_width=24  assert_rate=off  rate_source=Explicitly  period=1  output_port=on  block_type=assert
  assert_ts : xbsIndex_r4/Assert  assert_type=on  type_source=Explicitly  gui_display_data_type=Fixed-point  arith_type=Unsigned  n_bits=32  bin_pt=0  preci_type=Single  exp_width=8  frac_width=24  assert_rate=off  rate_source=Explicitly  period=1  output_port=on  block_type=assert
  assert_valid : xbsIndex_r4/Assert  assert_type=on  type_source=Explicitly  gui_display_data_type=Boolean  arith_type=Boolean  n_bits=1  bin_pt=0  preci_type=Single  exp_width=8  frac_width=24  assert_rate=off  rate_source=Explicitly  period=1  output_port=on  block_type=assert
  buscreate : Subsystem  AncestorBlock=casper_library_flow_control/bus_create  mask(bus_create){inputNum=5}
      mask prompts: inputNum "Number of inputs:"
      mask init:
      | bus_create_init(gcb,...
      |     'inputNum', inputNum);
  ss : Subsystem  Tag=casper:snapshot  AncestorBlock=casper_library_scopes/snapshot  mask(snapshot){storage=bram, dram_dimm=2, dram_clock=250, nsamples=10, data_width=128, offset=on, circap=off, value=off, ext_arm=off, ext_circ=off, provide_outputs=off, use_dsp48=on}
      mask prompts: storage "Storage medium"; dram_dimm "DRAM dimm"; dram_clock "DRAM clock rate"; nsamples "Number of Samples (2^?)"; data_width "Data width"; offset "Start delay support"; circap "Circular capture support"; value "Extra value capture support"; ext_arm "External arm support"; ext_circ "External circular capture support"; provide_outputs "Provide outputs"; use_dsp48 "Use DSP48s to implement counters"
      mask help:
      | Standard snap block, but with the following optional extras;
      |  1) Optionally delay the fabric trigger by a user-specified number of valids.
      |  2) Capture continuously after a trigger until a stop pulse is received. Data is captured into BRAM continuously, with old data being overwritten until a stop command is received. Then stop capturing when memory is filled. This enables you to get some data before and some data after the stop pulse. Use the 'tr_en_cnt' register to determine where you are in your vector. 'Addr' register's MSb now indicates 'busy capturing'.
      |  3) Optionally capture a value on an input port to a register at the same time as the first data sample.
      |  4) Implement counters using DSP48Es to save resources.
      mask init: same as s_c107m32k_vlbi/snap_acc/ss
      settings: AttributesFormatString=|
      | 128 wide, 1024 deep
      | debugID: 37129890
      mask TypeOptions storage: bram | dram
      mask Callback storage: snapshot_callback();
      mask TypeOptions dram_dimm: 1 | 2 | 3 | 4
      mask TypeOptions dram_clock: 200 | 250 | 266 | 300 | 333
      mask TypeOptions data_width: 8 | 16 | 32 | 64 | 128
  arm_out : Outport
  wires:
  ss/1(arm_out) -> arm_out/1
  buscreate/1(bus_out) -> ss/1(din)
  in_data/1 -> assert_data/1
  assert_data/1 -> buscreate/1(in1)
  in_ts/1 -> assert_ts/1
  assert_ts/1 -> buscreate/2(in2)
  in_ld/1 -> assert_ld/1
  assert_ld/1 -> buscreate/3(in3)
  in_delay/1 -> assert_delay/1
  assert_delay/1 -> buscreate/4(in4)
  in_valid/1 -> assert_valid/1
  assert_valid/1 -> buscreate/5(in5)
  we/1 -> ss/2(we)
  trig/1 -> ss/3(trig)

== system s_c107m32k_vlbi/bs_delay1/time_gen_bs ==
  wr_sync_in : Inport
  wr_en : Inport  Port=2
  wr_val_in : Inport  Port=3
  rd_sync_in : Inport  Port=4
  rd_en : Inport  Port=5
  rd_misc_in : Inport  Port=6
  Constant : xbsIndex_r4/Constant  const=2^n_bits_period-1  gui_display_data_type=Fixed-point  arith_type=Unsigned  n_bits=n_bits_period  bin_pt=0  preci_type=Single  exp_width=8  frac_width=24  explicit_period=on  period=1  equ=P=C  opselect=C  inp2=PCIN>>17  opr=+  inp1=P  carry=CIN  dbl_ovrd=off  block_type=constant
  Delay : xbsIndex_r4/Delay  rst=off  infoeditControl=Selection of Reset will increase slice count due to use of real FFs and instead of SRLs  en=off  latency=1  reg_retiming=on  dbl_ovrd=off  block_type=delay
      settings: infoedit=Hardware notes: A delay line is a chain, each link of which is an SRL16 or SRL32 followed by a flip-flop.
  Delay1 : xbsIndex_r4/Delay  rst=off  infoeditControl=Selection of Reset will increase slice count due to use of real FFs and instead of SRLs  en=off  latency=1  reg_retiming=on  dbl_ovrd=off  block_type=delay
      settings: infoedit=Hardware notes: A delay line is a chain, each link of which is an SRL16 or SRL32 followed by a flip-flop.
  Delay2 : xbsIndex_r4/Delay  rst=on  infoeditControl=Selection of Reset will increase slice count due to use of real FFs and instead of SRLs  en=on  latency=1  reg_retiming=on  dbl_ovrd=off  block_type=delay
      settings: infoedit=Hardware notes: A delay line is a chain, each link of which is an SRL16 or SRL32 followed by a flip-flop.
  Delay3 : xbsIndex_r4/Delay  rst=off  infoeditControl=Selection of Reset will increase slice count due to use of real FFs and instead of SRLs  en=off  latency=1  reg_retiming=on  dbl_ovrd=off  block_type=delay
      settings: infoedit=Hardware notes: A delay line is a chain, each link of which is an SRL16 or SRL32 followed by a flip-flop.
  Delay4 : xbsIndex_r4/Delay  rst=on  infoeditControl=Selection of Reset will increase slice count due to use of real FFs and instead of SRLs  en=on  latency=1  reg_retiming=on  dbl_ovrd=off  block_type=delay
      settings: infoedit=Hardware notes: A delay line is a chain, each link of which is an SRL16 or SRL32 followed by a flip-flop.
  Inverter1 : xbsIndex_r4/Inverter  en=off  latency=0  dbl_ovrd=off  block_type=inv
  Inverter2 : xbsIndex_r4/Inverter  en=off  latency=0  dbl_ovrd=off  block_type=inv
  Logical : xbsIndex_r4/Logical  logical_function=AND  inputs=2  en=off  latency=0  precision=Full  arith_type=Unsigned  n_bits=16  bin_pt=0  align_bp=on  dbl_ovrd=off  block_type=logical
  Logical1 : xbsIndex_r4/Logical  logical_function=OR  inputs=2  en=off  latency=0  precision=Full  arith_type=Unsigned  n_bits=16  bin_pt=0  align_bp=on  dbl_ovrd=off  block_type=logical
  Logical2 : xbsIndex_r4/Logical  logical_function=AND  inputs=2  en=off  latency=1  precision=Full  arith_type=Unsigned  n_bits=16  bin_pt=0  align_bp=on  dbl_ovrd=off  block_type=logical
  Logical3 : xbsIndex_r4/Logical  logical_function=AND  inputs=2  en=off  latency=0  precision=Full  arith_type=Unsigned  n_bits=16  bin_pt=0  align_bp=on  dbl_ovrd=off  block_type=logical
  Register1 : xbsIndex_r4/Register  init=0  rst=off  en=on  dbl_ovrd=off  block_type=register
  Relational : xbsIndex_r4/Relational  mode=a=b  op_type=Bool  en=off  latency=0  dbl_ovrd=off  block_type=relational
  counter : xbsIndex_r4/Counter  cnt_type=Free Running  cnt_to=Inf  operation=Up  start_count=0  cnt_by_val=2^n_bits_increment  arith_type=Unsigned  n_bits=n_bits_counter  bin_pt=0  load_pin=on  rst=off  en=on  explicit_period=on  period=1  use_behavioral_HDL=on  implementation=Fabric  dbl_ovrd=off  block_type=counter
  period : xbsIndex_r4/Counter  cnt_type=Free Running  cnt_to=Inf  operation=Up  start_count=0  cnt_by_val=1  arith_type=Unsigned  n_bits=n_bits_period  bin_pt=0  load_pin=off  rst=on  en=on  explicit_period=on  period=1  use_behavioral_HDL=off  implementation=Fabric  dbl_ovrd=off  block_type=counter
  rd_sync_out : Outport
  rd_dvalid : Outport  Port=2
  rd_val_out : Outport  Port=3
  rd_misc_out : Outport  Port=4
  wires:
  Logical3/1 -> counter/1, Logical1/1
  Register1/1 -> counter/2
  rd_en/1 -> Logical3/2, Delay4/1, Delay4/3, period/2, Logical2/2, Delay/1
  Inverter2/1 -> Logical3/1
  Delay4/1 -> Inverter2/1
  Logical2/1 -> Logical1/2
  rd_sync_in/1 -> period/1, Delay4/2, Delay1/1
  wr_val_in/1 -> Register1/1
  Delay3/1 -> rd_misc_out/1
  Delay1/1 -> rd_sync_out/1
  Delay/1 -> rd_dvalid/1
  rd_misc_in/1 -> Delay3/1
  Logical/1 -> Register1/2
  wr_en/1 -> Logical/2, Delay2/3, Delay2/1
  wr_sync_in/1 -> Delay2/2
  Logical1/1 -> counter/3
  Inverter1/1 -> Logical/1
  Relational/1 -> Logical2/1
  Constant/1 -> Relational/2
  period/1 -> Relational/1
  Delay2/1 -> Inverter1/1
  counter/1 -> rd_val_out/1

== system s_c107m32k_vlbi/calc_adc_sum_sq0/Subsystem5 ==
  din : Inport
  rst : Inport  Port=2
  max_check : xbsIndex_r4/Relational  mode=a>=b  op_type=Bool  en=off  latency=0  dbl_ovrd=off  block_type=relational
  max_reg : xbsIndex_r4/Register  init=0  rst=on  en=on  dbl_ovrd=off  block_type=register
      settings: xl_area=[0, 0, 0, 0, 0, 0, 0]
  max_reg1 : xbsIndex_r4/Register  init=0  rst=off  en=on  dbl_ovrd=off  block_type=register
      settings: xl_area=[0, 0, 0, 0, 0, 0, 0]
  max_reg2 : xbsIndex_r4/Register  init=0  rst=off  en=on  dbl_ovrd=off  block_type=register
      settings: xl_area=[0, 0, 0, 0, 0, 0, 0]
  min_check : xbsIndex_r4/Relational  mode=a<=b  op_type=Bool  en=off  latency=0  dbl_ovrd=off  block_type=relational
  min_reg : xbsIndex_r4/Register  init=0  rst=on  en=on  dbl_ovrd=off  block_type=register
      settings: xl_area=[0, 0, 0, 0, 0, 0, 0]
  max : Outport
  min : Outport  Port=2
  wires:
  din/1 -> min_reg/1, min_check/1, max_reg/1, max_check/1
  min_reg/1 -> max_reg2/1, min_check/2
  max_reg/1 -> max_reg1/1, max_check/2
  max_check/1 -> max_reg/3
  min_check/1 -> min_reg/3
  rst/1 -> max_reg1/2, max_reg2/2, min_reg/2, max_reg/2
  max_reg1/1 -> max/1
  max_reg2/1 -> min/1

== system s_c107m32k_vlbi/calc_adc_sum_sq0/bus_expand3 ==
  bus_in : Inport
  reinterpret{1..8} (8 alike) : xbsIndex_r4/Reinterpret  force_arith_type=on  arith_type="Signed  (2's comp)"  force_bin_pt=on  bin_pt=9  block_type=reinterpret
  slice1 : xbsIndex_r4/Slice  nbits=10  boolean_output=off  mode=Upper Bit Location + Width  bit1=-70  base1=MSB of Input  bit0=0  base0=LSB of Input  dbl_ovrd=off  block_type=slice
  slice2 : xbsIndex_r4/Slice  nbits=10  boolean_output=off  mode=Upper Bit Location + Width  bit1=-60  base1=MSB of Input  bit0=0  base0=LSB of Input  dbl_ovrd=off  block_type=slice
  slice3 : xbsIndex_r4/Slice  nbits=10  boolean_output=off  mode=Upper Bit Location + Width  bit1=-50  base1=MSB of Input  bit0=0  base0=LSB of Input  dbl_ovrd=off  block_type=slice
  slice4 : xbsIndex_r4/Slice  nbits=10  boolean_output=off  mode=Upper Bit Location + Width  bit1=-40  base1=MSB of Input  bit0=0  base0=LSB of Input  dbl_ovrd=off  block_type=slice
  slice5 : xbsIndex_r4/Slice  nbits=10  boolean_output=off  mode=Upper Bit Location + Width  bit1=-30  base1=MSB of Input  bit0=0  base0=LSB of Input  dbl_ovrd=off  block_type=slice
  slice6 : xbsIndex_r4/Slice  nbits=10  boolean_output=off  mode=Upper Bit Location + Width  bit1=-20  base1=MSB of Input  bit0=0  base0=LSB of Input  dbl_ovrd=off  block_type=slice
  slice7 : xbsIndex_r4/Slice  nbits=10  boolean_output=off  mode=Upper Bit Location + Width  bit1=-10  base1=MSB of Input  bit0=0  base0=LSB of Input  dbl_ovrd=off  block_type=slice
  slice8 : xbsIndex_r4/Slice  nbits=10  boolean_output=off  mode=Upper Bit Location + Width  bit1=0  base1=MSB of Input  bit0=0  base0=LSB of Input  dbl_ovrd=off  block_type=slice
  msb_out8 : Outport
  out7 : Outport  Port=2
  out6 : Outport  Port=3
  out5 : Outport  Port=4
  out4 : Outport  Port=5
  out3 : Outport  Port=6
  out2 : Outport  Port=7
  lsb_out1 : Outport  Port=8
  wires:
  bus_in/1 -> slice8/1, slice7/1, slice6/1, slice5/1, slice4/1, slice3/1, slice2/1, slice1/1
  slice8/1 -> reinterpret8/1
  reinterpret8/1 -> msb_out8/1
  slice7/1 -> reinterpret7/1
  reinterpret7/1 -> out7/1
  slice6/1 -> reinterpret6/1
  reinterpret6/1 -> out6/1
  slice5/1 -> reinterpret5/1
  reinterpret5/1 -> out5/1
  slice4/1 -> reinterpret4/1
  reinterpret4/1 -> out4/1
  slice3/1 -> reinterpret3/1
  reinterpret3/1 -> out3/1
  slice2/1 -> reinterpret2/1
  reinterpret2/1 -> out2/1
  slice1/1 -> reinterpret1/1
  reinterpret1/1 -> lsb_out1/1

== system s_c107m32k_vlbi/calc_adc_sum_sq0/negedge ==
  In : Inport
  Convert : xbsIndex_r4/Convert  gui_display_data_type=Fixed-point  arith_type=Boolean  n_bits=8  bin_pt=6  float_type=Single  exp_bits=8  fraction_bits=24  quantization=Truncate  overflow=Wrap  en=off  latency=0  pipeline=off  dbl_ovrd=off  block_type=convert
      settings: xl_area=[0, 0, 0, 0, 0, 0, 0]  block_version=10.1.3
  Delay : xbsIndex_r4/Delay  rst=off  infoeditControl=Selection of Reset will increase slice count due to use of real FFs and instead of SRLs  en=off  latency=1  reg_retiming=off  dbl_ovrd=off  block_type=delay
      settings: xl_area=[0, 0, 0, 0, 0, 0, 0]
  Inverter1 : xbsIndex_r4/Inverter  en=off  latency=0  dbl_ovrd=off  block_type=inv
      settings: xl_area=[0, 0, 0, 0, 0, 0, 0]
  Logical : xbsIndex_r4/Logical  logical_function=AND  inputs=2  en=off  latency=0  precision=Full  arith_type=Unsigned  n_bits=8  bin_pt=2  align_bp=on  dbl_ovrd=off  block_type=logical
      settings: xl_area=[0, 0, 0, 0, 0, 0, 0]
  Out1 : Outport
  wires:
  Convert/1 -> Out1/1
  Delay/1 -> Logical/1
  In/1 -> Delay/1, Inverter1/1
  Logical/1 -> Convert/1
  Inverter1/1 -> Logical/2

== system s_c107m32k_vlbi/calc_adc_sum_sq1/Subsystem5 ==
  din : Inport
  rst : Inport  Port=2
  max_check : xbsIndex_r4/Relational  mode=a>=b  op_type=Bool  en=off  latency=0  dbl_ovrd=off  block_type=relational
  max_reg : xbsIndex_r4/Register  init=0  rst=on  en=on  dbl_ovrd=off  block_type=register
      settings: xl_area=[0, 0, 0, 0, 0, 0, 0]
  max_reg1 : xbsIndex_r4/Register  init=0  rst=off  en=on  dbl_ovrd=off  block_type=register
      settings: xl_area=[0, 0, 0, 0, 0, 0, 0]
  max_reg2 : xbsIndex_r4/Register  init=0  rst=off  en=on  dbl_ovrd=off  block_type=register
      settings: xl_area=[0, 0, 0, 0, 0, 0, 0]
  min_check : xbsIndex_r4/Relational  mode=a<=b  op_type=Bool  en=off  latency=0  dbl_ovrd=off  block_type=relational
  min_reg : xbsIndex_r4/Register  init=0  rst=on  en=on  dbl_ovrd=off  block_type=register
      settings: xl_area=[0, 0, 0, 0, 0, 0, 0]
  max : Outport
  min : Outport  Port=2
  wires:
  max_reg2/1 -> min/1
  max_reg1/1 -> max/1
  rst/1 -> max_reg/2, min_reg/2, max_reg2/2, max_reg1/2
  min_check/1 -> min_reg/3
  max_check/1 -> max_reg/3
  max_reg/1 -> max_check/2, max_reg1/1
  min_reg/1 -> min_check/2, max_reg2/1
  din/1 -> max_check/1, max_reg/1, min_check/1, min_reg/1

== system s_c107m32k_vlbi/calc_adc_sum_sq1/bus_expand3 ==
  bus_in : Inport
  reinterpret{1..8} (8 alike) : xbsIndex_r4/Reinterpret  force_arith_type=on  arith_type="Signed  (2's comp)"  force_bin_pt=on  bin_pt=9  block_type=reinterpret
  slice1 : xbsIndex_r4/Slice  nbits=10  boolean_output=off  mode=Upper Bit Location + Width  bit1=-70  base1=MSB of Input  bit0=0  base0=LSB of Input  dbl_ovrd=off  block_type=slice
  slice2 : xbsIndex_r4/Slice  nbits=10  boolean_output=off  mode=Upper Bit Location + Width  bit1=-60  base1=MSB of Input  bit0=0  base0=LSB of Input  dbl_ovrd=off  block_type=slice
  slice3 : xbsIndex_r4/Slice  nbits=10  boolean_output=off  mode=Upper Bit Location + Width  bit1=-50  base1=MSB of Input  bit0=0  base0=LSB of Input  dbl_ovrd=off  block_type=slice
  slice4 : xbsIndex_r4/Slice  nbits=10  boolean_output=off  mode=Upper Bit Location + Width  bit1=-40  base1=MSB of Input  bit0=0  base0=LSB of Input  dbl_ovrd=off  block_type=slice
  slice5 : xbsIndex_r4/Slice  nbits=10  boolean_output=off  mode=Upper Bit Location + Width  bit1=-30  base1=MSB of Input  bit0=0  base0=LSB of Input  dbl_ovrd=off  block_type=slice
  slice6 : xbsIndex_r4/Slice  nbits=10  boolean_output=off  mode=Upper Bit Location + Width  bit1=-20  base1=MSB of Input  bit0=0  base0=LSB of Input  dbl_ovrd=off  block_type=slice
  slice7 : xbsIndex_r4/Slice  nbits=10  boolean_output=off  mode=Upper Bit Location + Width  bit1=-10  base1=MSB of Input  bit0=0  base0=LSB of Input  dbl_ovrd=off  block_type=slice
  slice8 : xbsIndex_r4/Slice  nbits=10  boolean_output=off  mode=Upper Bit Location + Width  bit1=0  base1=MSB of Input  bit0=0  base0=LSB of Input  dbl_ovrd=off  block_type=slice
  msb_out8 : Outport
  out7 : Outport  Port=2
  out6 : Outport  Port=3
  out5 : Outport  Port=4
  out4 : Outport  Port=5
  out3 : Outport  Port=6
  out2 : Outport  Port=7
  lsb_out1 : Outport  Port=8
  wires:
  bus_in/1 -> slice8/1, slice7/1, slice6/1, slice5/1, slice4/1, slice3/1, slice2/1, slice1/1
  slice8/1 -> reinterpret8/1
  reinterpret8/1 -> msb_out8/1
  slice7/1 -> reinterpret7/1
  reinterpret7/1 -> out7/1
  slice6/1 -> reinterpret6/1
  reinterpret6/1 -> out6/1
  slice5/1 -> reinterpret5/1
  reinterpret5/1 -> out5/1
  slice4/1 -> reinterpret4/1
  reinterpret4/1 -> out4/1
  slice3/1 -> reinterpret3/1
  reinterpret3/1 -> out3/1
  slice2/1 -> reinterpret2/1
  reinterpret2/1 -> out2/1
  slice1/1 -> reinterpret1/1
  reinterpret1/1 -> lsb_out1/1

== system s_c107m32k_vlbi/calc_adc_sum_sq1/negedge ==
  In : Inport
  Convert : xbsIndex_r4/Convert  gui_display_data_type=Fixed-point  arith_type=Boolean  n_bits=8  bin_pt=6  float_type=Single  exp_bits=8  fraction_bits=24  quantization=Truncate  overflow=Wrap  en=off  latency=0  pipeline=off  dbl_ovrd=off  block_type=convert
      settings: xl_area=[0, 0, 0, 0, 0, 0, 0]  block_version=10.1.3
  Delay : xbsIndex_r4/Delay  rst=off  infoeditControl=Selection of Reset will increase slice count due to use of real FFs and instead of SRLs  en=off  latency=1  reg_retiming=off  dbl_ovrd=off  block_type=delay
      settings: xl_area=[0, 0, 0, 0, 0, 0, 0]
  Inverter1 : xbsIndex_r4/Inverter  en=off  latency=0  dbl_ovrd=off  block_type=inv
      settings: xl_area=[0, 0, 0, 0, 0, 0, 0]
  Logical : xbsIndex_r4/Logical  logical_function=AND  inputs=2  en=off  latency=0  precision=Full  arith_type=Unsigned  n_bits=8  bin_pt=2  align_bp=on  dbl_ovrd=off  block_type=logical
      settings: xl_area=[0, 0, 0, 0, 0, 0, 0]
  Out1 : Outport
  wires:
  Inverter1/1 -> Logical/2
  Logical/1 -> Convert/1
  In/1 -> Inverter1/1, Delay/1
  Delay/1 -> Logical/1
  Convert/1 -> Out1/1

== system s_c107m32k_vlbi/calc_ddc_pwr0/negedge ==
  In : Inport
  Convert : xbsIndex_r4/Convert  gui_display_data_type=Fixed-point  arith_type=Boolean  n_bits=8  bin_pt=6  float_type=Single  exp_bits=8  fraction_bits=24  quantization=Truncate  overflow=Wrap  en=off  latency=0  pipeline=off  dbl_ovrd=off  block_type=convert
      settings: xl_area=[0, 0, 0, 0, 0, 0, 0]  block_version=10.1.3
  Delay : xbsIndex_r4/Delay  rst=off  infoeditControl=Selection of Reset will increase slice count due to use of real FFs and instead of SRLs  en=off  latency=1  reg_retiming=off  dbl_ovrd=off  block_type=delay
      settings: xl_area=[0, 0, 0, 0, 0, 0, 0]
  Inverter1 : xbsIndex_r4/Inverter  en=off  latency=0  dbl_ovrd=off  block_type=inv
      settings: xl_area=[0, 0, 0, 0, 0, 0, 0]
  Logical : xbsIndex_r4/Logical  logical_function=AND  inputs=2  en=off  latency=0  precision=Full  arith_type=Unsigned  n_bits=8  bin_pt=2  align_bp=on  dbl_ovrd=off  block_type=logical
      settings: xl_area=[0, 0, 0, 0, 0, 0, 0]
  Out1 : Outport
  wires:
  Convert/1 -> Out1/1
  Delay/1 -> Logical/1
  In/1 -> Delay/1, Inverter1/1
  Logical/1 -> Convert/1
  Inverter1/1 -> Logical/2
